simulink model "AllSystemInLoop"  (R2025b)
settings: Solver=ode4  StartTime=0.0  StopTime=inf  FixedStep=0.01  RelTol=1e-3
InitFcn:
  | load("pre-design_data")
undefined symbols (not defined in the file or in its folder): DiscIntNeverNeededParam
libraries: ASEToolBox x11, simulink x1
settings Model: Creator=admin  LastModifiedBy=zqhkd
settings DataIOCC: SaveFinalState=on  SaveOutput=off  InspectSignalLogs=on  SaveTime=off
settings OptimizationCC: EnhancedBackFolding=on  PassReuseOutputArgsAs=Individual arguments  ZeroExternalMemoryAtStartup=off  ZeroInternalMemoryAtStartup=off  OptimizeBlockOrder=speed  DifferentSizesBufferReuse=on  OptimizationCustomize=off  EfficientTunableParamExpr=on
settings DebuggingCC: ParameterTunabilityLossMsg=error
settings HardwareCC: ProdBitPerLong=64.0  ProdHWDeviceType=Intel->x86-64 (Linux 64)
settings SFSimCC: MATLABDynamicMemAlloc=off
settings RTWCC: SystemTargetFile=ert.tlc  TemplateMakefile=ert_default_tmf  RetainRTWFile=on  Toolchain=Microsoft Visual C++ 2022 v17.0 | nmake (64-bit Windows)  GPUComputeCapability=3.5  Description=Embedded Coder
settings CodeAppCC: ForceParamTrailComments=on  IgnoreCustomStorageClasses=off  OperatorAnnotations=on  SimulinkDataObjDesc=on  SFDataObjDesc=on  InsertBlockDesc=on
settings ERTTargetCC: InlinedParameterPlacement=Hierarchical  RTWCAPISignals=on  RTWCAPIParams=on  RTWCAPIStates=on  RTWCAPIRootIO=on  ERTCustomFileTemplate=example_file_process.tlc  DynamicArrayContainerType=coder::array  TargetLangStandard=C99 (ISO)  SupportContinuousTime=on

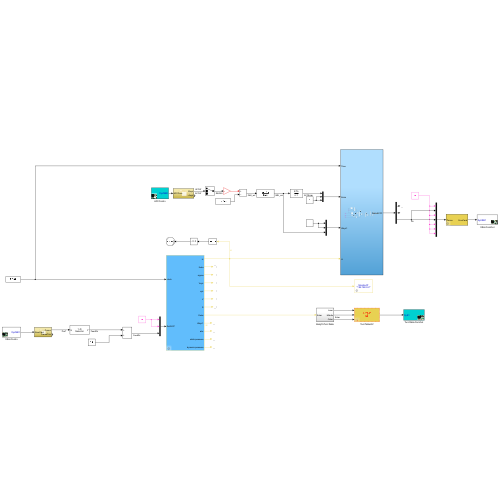
[thumbnail: Simulink's stored preview of the top-level diagram]
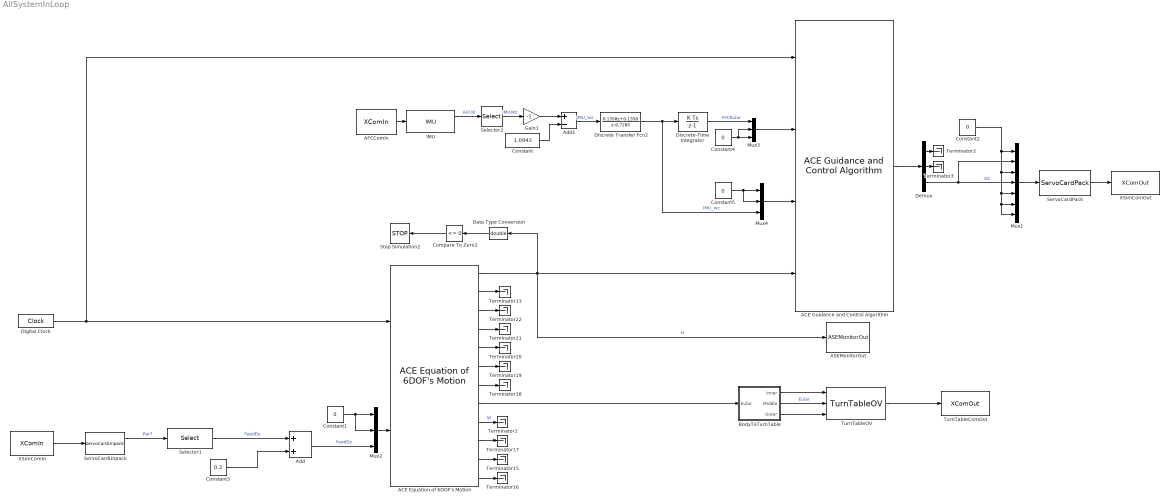
== system AllSystemInLoop ==
  ACE Equation of 6DOF's Motion : ASEToolBox/Aerocraft Model/ACE Equation of 6DOF's Motion
      settings: SourceProductName=ASEToolBox
  ACE Guidance and Control Algorithm : ASEToolBox/Aerocraft Model/ACE Guidance and Control Algorithm  SystemSampleTime=-1  VariantActivationTime=update diagram  EmptyChoice=off  PassThrough=off  PassThroughVariantControl=(default)  EmptyChoiceVariantControl=(default)  AllowFlexibleInterface=on  Latency=0  AutoFrameSizeCalculation=off
      settings: SourceProductName=ASEToolBox
  AFCComIn : ASEToolBox/COMModule/XComIn  g_serial_select=ttyUSB0  g_baudrate=460800  g_parity=None  g_databit=8  g_stopbit=1  g_data_size=6*4+12  g_sample_time=0.01
      settings: SourceProductName=ASEToolBox
  ASEMonitorOut : ASEToolBox/SIMSystemModule/ASEMonitorOut  Tag=ASEMonitorOutTag  g_iVarNum=1  g_iFrameType=10  g_hostIP="\"192.168.0.2\""
      settings: SourceProductName=ASEToolBox
  Add : Sum
  Add1 : Sum  Inputs=+-
  BodyToTurnTable : Subsystem
  Compare To Zero2 : simulink/Logic and Bit Operations/Compare To Zero  relop=<=  OutDataTypeStr=boolean
  Constant : Constant  Value=1.0943
  Constant{1..2,4..5} (4 alike) : Constant  Value=0
  Constant3 : Constant  Value=0.2
  Data Type Conversion : DataTypeConversion  OutDataTypeStr=double  SaturateOnIntegerOverflow=off  RndMeth=Floor
  Demux : Demux  Outputs=3
  Digital Clock : DigitalClock  SampleTime=0.01
  Discrete Transfer Fcn2 : DiscreteTransferFcn  Numerator=[0.1358 0.1358]  Denominator=[1 -0.7285]
  Discrete-Time Integrator : DiscreteIntegrator  InitialCondition=60  SampleTime=-1  ICPrevOutput=DiscIntNeverNeededParam  ICPrevScaledInput=DiscIntNeverNeededParam
  Gain1 : Gain  Gain=-1
  IMU : ASEToolBox/ACEModule/IMU  SystemSampleTime=-1  VariantActivationTime=update diagram  EmptyChoice=off  PassThrough=off  PassThroughVariantControl=(default)  EmptyChoiceVariantControl=(default)  AllowFlexibleInterface=on  Latency=0  AutoFrameSizeCalculation=off
      settings: SourceProductName=ASEToolBox
  Mux1 : Mux  Inputs=7
  Mux2 : Mux  Inputs=3
  Mux3 : Mux  Inputs=3
  Mux4 : Mux  Inputs=3
  Selector1 : Selector  InputPortWidth=7  IndexOptions=Index vector (dialog)  Indices=2  OutputSizes=1
  Selector2 : Selector  InputPortWidth=3  IndexOptions=Index vector (dialog)  Indices=1  OutputSizes=1
  ServoCardPack : ASEToolBox/ACEModule/ServoCardPack  g_FrameType=80  g_SendId=0
      settings: SourceProductName=ASEToolBox
  ServoCardUnpack : ASEToolBox/ACEModule/ServoCardUnpack  SystemSampleTime=-1  VariantActivationTime=update diagram  EmptyChoice=off  PassThrough=off  PassThroughVariantControl=(default)  EmptyChoiceVariantControl=(default)  AllowFlexibleInterface=on  Latency=0  AutoFrameSizeCalculation=off
      settings: SourceProductName=ASEToolBox
  Stop Simulation2 : Stop
  Terminator{1..3,13,15..22} (12 alike) : Terminator
  TurnTableComOut : ASEToolBox/COMModule/XComOut  g_serial_select=ttyS1  g_baudrate=115200  g_parity=None  g_databit=8  g_stopbit=1  g_sample_time=0.01
      settings: SourceProductName=ASEToolBox
  TurnTableOV : ASEToolBox/ACEModule/TurnTableOV  SystemSampleTime=-1  VariantActivationTime=update diagram  Latency=0  AutoFrameSizeCalculation=off
      settings: SourceProductName=ASEToolBox
  XSimComIn : ASEToolBox/COMModule/XComIn  g_serial_select=ttyUSB1  g_baudrate=460800  g_parity=None  g_databit=8  g_stopbit=1  g_data_size=12+7*4  g_sample_time=0.01
      settings: SourceProductName=ASEToolBox
  XSimComOut : ASEToolBox/COMModule/XComOut  g_serial_select=ttyUSB1  g_baudrate=460800  g_parity=None  g_databit=8  g_stopbit=1  g_sample_time=0.01
      settings: SourceProductName=ASEToolBox
  wires:
  ACE Equation of 6DOF's Motion/11 -> Terminator15/1
  ACE Equation of 6DOF's Motion/3 -> Terminator22/1
  ACE Equation of 6DOF's Motion/7 -> Terminator18/1
  ACE Equation of 6DOF's Motion/2 -> Terminator13/1
  ACE Equation of 6DOF's Motion/12 -> Terminator16/1
  ACE Equation of 6DOF's Motion/1 -> ASEMonitorOut/1, Data Type Conversion/1, ACE Guidance and Control Algorithm/4  "H"
  ACE Equation of 6DOF's Motion/4 -> Terminator21/1
  Compare To Zero2/1 -> Stop Simulation2/1
  ACE Equation of 6DOF's Motion/6 -> Terminator19/1
  Digital Clock/1 -> ACE Equation of 6DOF's Motion/1, ACE Guidance and Control Algorithm/1
  ACE Equation of 6DOF's Motion/5 -> Terminator20/1
  ACE Equation of 6DOF's Motion/10 -> Terminator17/1
  Data Type Conversion/1 -> Compare To Zero2/1
  BodyToTurnTable/1(Inner) -> TurnTableOV/1
  BodyToTurnTable/2(Middle) -> TurnTableOV/2  "Eular"
  BodyToTurnTable/3(Outer) -> TurnTableOV/3
  IMU/1 -> Selector2/1  "AFCW"
  Constant2/1 -> Mux1/7, Mux1/6, Mux1/5, Mux1/3, Mux1/1
  Demux/3 -> Mux1/2, Mux1/4  "Dz"
  ServoCardUnpack/1 -> Selector1/1  "Par7"
  Mux2/1 -> ACE Equation of 6DOF's Motion/2
  Constant1/1 -> Mux2/2, Mux2/1
  ACE Guidance and Control Algorithm/1 -> Demux/1
  Selector1/1 -> Add/1  "FeedDz"
  Constant3/1 -> Add/2
  XSimComIn/1 -> ServoCardUnpack/1
  ServoCardPack/1 -> XSimComOut/1
  Mux1/1 -> ServoCardPack/1
  AFCComIn/1 -> IMU/1
  TurnTableOV/1 -> TurnTableComOut/1
  Add/1 -> Mux2/3  "FeedDz"
  Selector2/1 -> Gain1/1  "IMUWz"
  Add1/1 -> Discrete Transfer Fcn2/1  "IMU_wz"
  Discrete-Time Integrator/1 -> Mux3/1  "AFCEular"
  Gain1/1 -> Add1/1
  Constant/1 -> Add1/2
  Mux3/1 -> ACE Guidance and Control Algorithm/2
  Constant4/1 -> Mux3/2, Mux3/3
  Mux4/1 -> ACE Guidance and Control Algorithm/3
  Constant5/1 -> Mux4/1, Mux4/2
  ACE Equation of 6DOF's Motion/8 -> BodyToTurnTable/1(Eular)
  ACE Equation of 6DOF's Motion/9 -> Terminator1/1  "W"
  Discrete Transfer Fcn2/1 -> Mux4/3, Discrete-Time Integrator/1  "IMU_wz"
  Demux/1 -> Terminator2/1
  Demux/2 -> Terminator3/1

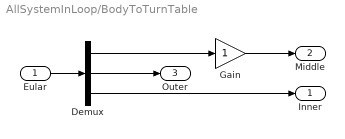
== system AllSystemInLoop/BodyToTurnTable ==
  Eular : Inport
  Demux : Demux  Outputs=3
  Gain : Gain
  Inner : Outport
  Middle : Outport  Port=2
  Outer : Outport  Port=3
  wires:
  Demux/1 -> Gain/1
  Eular/1 -> Demux/1
  Gain/1 -> Middle/1
  Demux/3 -> Inner/1
  Demux/2 -> Outer/1
